simulink model "DRLHevIps"  (R2025b)
settings: Solver=ode23tb  StartTime=0  StopTime=stop_time+1  FixedStep=ts  RelTol=1e-3  AbsTol=1e-4
model workspace (MAT data in the model file):
  BattChrgMax : Simulink.Parameter (value not decoded)
  BattDischrgMax : Simulink.Parameter (value not decoded)
  BrkPrsMax : Simulink.Parameter (value not decoded)
  DiffRatio : Simulink.Parameter (value not decoded)
  EVSpdLmt : Simulink.Parameter (value not decoded)
  EngIdle : Simulink.Parameter (value not decoded)
  EngPwr : Simulink.Parameter (value not decoded)
  EngSpd : Simulink.Parameter (value not decoded)
  EngTrq : Simulink.Parameter (value not decoded)
  EngTrqWhl : Simulink.Parameter (value not decoded)
  GenMapEff : Simulink.Parameter (value not decoded)
  GenMapSpdIndex : Simulink.Parameter (value not decoded)
  GenMapTrqIndex : Simulink.Parameter (value not decoded)
  GenPwrMax : Simulink.Parameter (value not decoded)
  GenSpd : Simulink.Parameter (value not decoded)
  GenTrq : Simulink.Parameter (value not decoded)
  GenTrqMax : Simulink.Parameter (value not decoded)
  MotMapEff : Simulink.Parameter (value not decoded)
  MotMapSpdIndex : Simulink.Parameter (value not decoded)
  MotMapTrqIndex : Simulink.Parameter (value not decoded)
  MotPwr : Simulink.Parameter (value not decoded)
  MotSpd : Simulink.Parameter (value not decoded)
  MotTrq : Simulink.Parameter (value not decoded)
  Ndiff : Simulink.Parameter (value not decoded)
  Nr1 : Simulink.Parameter (value not decoded)
  Nr2 : Simulink.Parameter (value not decoded)
  Ns1 : Simulink.Parameter (value not decoded)
  Ns2 : Simulink.Parameter (value not decoded)
  NsysWhl : Simulink.Parameter (value not decoded)
  SOCChrgFactor : Simulink.Parameter (value not decoded)
  SOCerr : Simulink.Parameter (value not decoded)
  SOCmax : Simulink.Parameter (value not decoded)
  SOCmin : Simulink.Parameter (value not decoded)
  SOCtarget : Simulink.Parameter (value not decoded)
  SysTrqWhl : Simulink.Parameter (value not decoded)
  k : Simulink.Parameter (value not decoded)
values from neighbouring files (symbols this model uses):
  cyc_time = WLTC(:,1)    [mdlrun_time_DG.m]
  cyc_vel = WLTC(:,2)    [mdlrun_time_DG.m]
  en_actsmo = 1    [mdlrun_time_DG.m]
  en_elec = 1    [mdlrun_time_DG.m]
  en_gas = 1    [mdlrun_time_DG.m]
  en_SOCpen = 1    [mdlrun_time_DG.m]
  k_actsmo = 5e-2    (= 0.05)    [mdlrun_time_DG.m]
  k_elec = 1    [mdlrun_time_DG.m]
  k_gas = 1    [mdlrun_time_DG.m]
  k_SOCpen = 1.2    [mdlrun_time_DG.m]
  obs_max = 1e4*[0.0020, 0.0090, 0.0100, 0.0100, 8.4000, 0.0100,                0.0056, 0.1011, 2.8000,      0, 0.0001, 0.0132,                0.0740, 2.6065, 0.0339, 0.0949, 0.0117, 2.4444]    [mdlrun_time_DG.m]
  obs_min = 1e4*[0.0010, 0.0070,      0,      0, 0.8400,      0,                     0, -0.0005,     0, -2.8000,     0, -0.0032               -0.0694, -2.7092, -0.0030,    0, -0.0001, -2.7647]    [mdlrun_time_DG.m]
  Price_elec = 1    [mdlrun_time_DG.m]
  Price_gas = 7.14    [mdlrun_time_DG.m]
  rho_gas = 0.739    [mdlrun_time_DG.m]
  stop_time = cyc_time(end)    [mdlrun_time_DG.m]
  ts = 1    [mdlrun_time_DG.m]
symbols that are objects in the model workspace (value not decoded): BattChrgMax, BattDischrgMax, BrkPrsMax, DiffRatio, EngIdle, EngPwr, EngSpd, EngTrq, EngTrqWhl, EVSpdLmt, GenMapSpdIndex, GenMapTrqIndex, GenPwrMax, GenSpd, GenTrq, GenTrqMax, k, MotMapSpdIndex, MotMapTrqIndex, MotPwr, MotSpd, MotTrq, Ndiff, Nr1, Nr2, Ns1, Ns2, NsysWhl, SOCChrgFactor, SOCerr, SOCmin, SOCtarget, SysTrqWhl
undefined symbols (not defined in the file or in its folder): n_ool, T_ool
libraries: simulink x29, autolibutils x6, slpidlib x2, rllib x2, SignalEditorBlockLib x1, autolibshared x1, autolibhevctrlrcommon x1
(part 3 of 4)

== system DRLHevIps/xCU/xCU/VCU/DRL_Based2_0/DRL action Handle ==
  action : Inport
  EngSpdFdbk : Inport  Port=2
  WhlTrqCmd : Inport  Port=3
  1-D Lookup Table1 : Lookup_n-D  NumberOfTableDimensions=1  BreakpointsForDimension1=[-1, 1]  Table=[n_ool(1), n_ool(end)]  InternalRulePriority=Speed  RndMeth=Simplest
      settings: AttributesFormatString=|
      | %<BreakpointsForDimension1>
      | %<Table>
  1-D Lookup Table2 : Lookup_n-D  NumberOfTableDimensions=1  BreakpointsForDimension1=n_ool  Table=T_ool  InternalRulePriority=Speed  RndMeth=Simplest
      settings: AttributesFormatString=|
      | %<BreakpointsForDimension1>
      | %<Table>
  1-D Lookup Table3 : Lookup_n-D  Commented=on  NumberOfTableDimensions=1  BreakpointsForDimension1=[-1, 1]  Table=[0, max(EngPwr(1,1:15))]  InternalRulePriority=Speed  RndMeth=Simplest
      settings: AttributesFormatString=|
      | %<BreakpointsForDimension1>
      | %<Table>
  Add : Sum  Inputs=-+
  Add1 : Sum
  Add2 : Sum  Inputs=+-
  Gain : Gain  Gain=1/DiffRatio
  Gain1 : Gain  Gain=1/(Nr2/Ns2)
  OptimalEngineSpeed : Lookup_n-D  Commented=on  NumberOfTableDimensions=1  BreakpointsForDimension1=[0 EngPwr(1,1:15)]  Table=[EngIdle*30/pi EngSpd(1,1:15)]  ExtrapMethod=Clip  UseLastTableValue=on  InternalRulePriority=Speed  RndMeth=Simplest
      settings: AttributesFormatString=|
      | %<BreakpointsForDimension1>
      | %<Table>
  OptimalEngineTorque : Lookup_n-D  Commented=on  NumberOfTableDimensions=1  BreakpointsForDimension1=[0 EngPwr(1,1:15)]  Table=[0 EngTrq(1,1:15)]  ExtrapMethod=Clip  UseLastTableValue=on  InternalRulePriority=Speed  RndMeth=Simplest
      settings: AttributesFormatString=|
      | %<BreakpointsForDimension1>
      | %<Table>
  PID Controller : slpidlib/PID Controller  Controller=PI  Form=Parallel  TimeDomain=Discrete-time  UseExternalTs=off  SampleTime=-1  IntegratorMethod=Forward Euler  FilterMethod=Forward Euler  ControllerParametersSource=internal  P=0.18  I=1.0  UseKiTs=off  D=0  UseExternalDerivativeSource=off  N=100  UseFilter=on  TunerSelectOption=Transfer Function Based (PID Tuner App)  InitialConditionSource=internal  InitialConditionForIntegrator=0  InitialConditionForFilter=0  DifferentiatorICPrevScaledInput=0  ExternalReset=none  TrackingMode=off  Kt=1  LimitOutput=on  SatLimitsSource=internal  UpperSaturationLimit=207*42/60-20  LowerSaturationLimit=20-207*42/60  LinearizeAsGain=on  AntiWindupMode=clamping  Kb=1  LimitIntegrator=off  UpperIntegratorSaturationLimit=inf  LowerIntegratorSaturationLimit=-inf  POutMin=[]  POutMax=[]  IOutMin=[]  IOutMax=[]  DOutMin=[]  DOutMax=[]  NOutMin=[]  NOutMax=[]  SumOutMin=[]  SumOutMax=[]  SaturationOutMin=[]  SaturationOutMax=[]  PParamMin=[]  PParamMax=[]  IParamMin=[]  IParamMax=[]  DParamMin=[]  DParamMax=[]  NParamMin=[]  NParamMax=[]  KbParamMin=[]  KbParamMax=[]  KtParamMin=[]  KtParamMax=[]  KbOutMin=[]  KbOutMax=[]  KtOutMin=[]  KtOutMax=[]  IntegratorOutMin=[]  IntegratorOutMax=[]  FilterOutMin=[]  FilterOutMax=[]  SumI1OutMin=[]  SumI1OutMax=[]  SumI2OutMin=[]  SumI2OutMax=[]  SumI3OutMin=[]  SumI3OutMax=[]  SumI4OutMin=[]  SumI4OutMax=[]  SumDOutMin=[]  SumDOutMax=[]  DifferentiatorOutMin=[]  DifferentiatorOutMax=[]  FilterDiffOutCoefMin=[]  FilterDiffOutCoefMax=[]  ReciprocalOutMin=[]  ReciprocalOutMax=[]  SumDenOutMin=[]  SumDenOutMax=[]  SumNumOutMin=[]  SumNumOutMax=[]  DivideOutMin=[]  DivideOutMax=[]  UdiffTsProdOutMin=[]  UdiffTsProdOutMax=[]  NTsProdOutMin=[]  NTsProdOutMax=[]  UintegralTsProdOutMin=[]  UintegralTsProdOutMax=[]  UngainTsProdOutMin=[]  UngainTsProdOutMax=[]  ClampingZeroOutDataTypeStr=Inherit: Inherit via back propagation  ClampingZeroOutMin=[]  ClampingZeroOutMax=[]  FilterDenConstantOutDataTypeStr=Inherit: Inherit via back propagation  FilterDenConstantOutMin=[]  FilterDenConstantOutMax=[]  PCopyOutDataTypeStr=Inherit: Inherit via back propagation  PCopyOutMin=[]  PCopyOutMax=[]  NCopyOutDataTypeStr=Inherit: Inherit via back propagation  NCopyOutMin=[]  NCopyOutMax=[]  IntegratorContinuousStateAttributes=''  IntegratorStateMustResolveToSignalObject=off  IntegratorRTWStateStorageClass=Auto  FilterContinuousStateAttributes=''  FilterStateMustResolveToSignalObject=off  FilterRTWStateStorageClass=Auto  ParallelPVariant=InternalParameters  IdealPVariant=Disabled  IVariant=InternalParameters  DVariant=Disabled  IntegratorVariant=Discrete  SatVariant=Enabled  AWVariant=DiscClampingParallel  PCopyVariant=Disabled  TRVariant=Disabled  FdbkBlocksVariant=Forward  IdealPFdbkVariant=Disabled  SatFdbkVariant=Disabled  DerivativeFilterVariant=Disabled  NVariant=Disabled  NCopyVariant=Disabled_SignalSpec  FilterICVariant=Disabled  IntegratorICVariant=InternalICs  ExternalResetVariant=Disabled  TRSumVariant=Passthrough  SumFdbkVariant=Disabled  SumVariant=Sum_PI  TsampFilterVariant=InternalTs  TsampNgainVariant=Passthrough  TsampIntegralVariant=Disabled_SignalSpec  ExternalSaturationOutDataTypeStr=Inherit: Same as second input  DerivativeSourceVariant=Disabled  PreIntVariant=InternalPreInt
  Product : Product
  Product1 : Product
  Saturation : Saturate  UpperLimit=207*42/60  LowerLimit=-207*42/60
  k1 : Constant  Value=-(1/(1+k))
  k2 : Constant  Value=k/(1+k)
  rads_to_rpm : Gain  Gain=30/pi
  EngTrqCmd : Outport
  GenTrqCmd : Outport  Port=2
  MotTrqCmd : Outport  Port=3
  wires:
  k1/1 -> Product/2
  Add1/1 -> Saturation/1
  WhlTrqCmd/1 -> Gain/1
  k2/1 -> Product1/2
  Product1/1 -> Add/1  "T_e_to_ring"
  Gain/1 -> Add/2  "T_req"
  Add/1 -> Gain1/1
  Product/1 -> Add1/1  "T_g_cmd"
  EngSpdFdbk/1 -> rads_to_rpm/1
  Add2/1 -> PID Controller/1
  PID Controller/1 -> Add1/2
  Saturation/1 -> GenTrqCmd/1
  Gain1/1 -> MotTrqCmd/1  "T_m_cmd"
  rads_to_rpm/1 -> Add2/2
  [EngTrqCmd] -> Product/1
  [EngSpdCmd] -> Add2/1
  [EngTrqCmd] -> Product1/1
  1-D Lookup Table1/1 -> 1-D Lookup Table2/1, [EngSpdCmd]  "w_e_cmd"
  action/1 -> 1-D Lookup Table1/1
  1-D Lookup Table3/1 -> OptimalEngineSpeed/1, OptimalEngineTorque/1
  1-D Lookup Table2/1 -> EngTrqCmd/1, [EngTrqCmd]

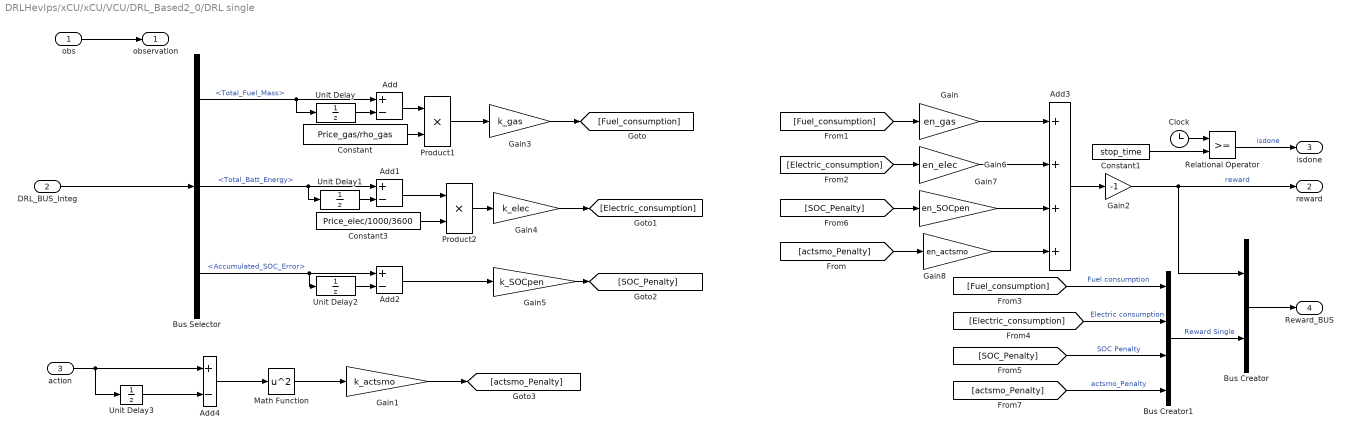
== system DRLHevIps/xCU/xCU/VCU/DRL_Based2_0/DRL single ==
  obs : Inport
  DRL_BUS_Integ : Inport  Port=2
  action : Inport  Port=3
  Add{,1..2,4} (4 alike) : Sum  Inputs=+-
  Add3 : Sum  Inputs=++++
  Bus Creator : BusCreator  Inputs=2
  Bus Creator1 : BusCreator  Inputs=4
  Bus Selector : BusSelector  OutputSignals=Total_Fuel_Mass,Total_Batt_Energy,Accumulated_SOC_Error
  Clock : Clock
  Constant : Constant  Value=Price_gas/rho_gas
  Constant1 : Constant  Value=stop_time
  Constant3 : Constant  Value=Price_elec/1000/3600
  Gain : Gain  Gain=en_gas
  Gain1 : Gain  Gain=k_actsmo
  Gain2 : Gain  Gain=-1
  Gain3 : Gain  Gain=k_gas
  Gain4 : Gain  Gain=k_elec
  Gain5 : Gain  Gain=k_SOCpen
  Gain6 : Gain  Gain=en_elec
  Gain7 : Gain  Gain=en_SOCpen
  Gain8 : Gain  Gain=en_actsmo
  Math Function : Math  Operator=square
  Product1 : Product
  Product2 : Product
  Relational Operator : RelationalOperator  OutDataTypeStr=boolean  RndMeth=Simplest  InputSameDT=off
  Unit Delay : UnitDelay  SampleTime=ts  HasFrameUpgradeWarning=on
  Unit Delay1 : UnitDelay  SampleTime=ts  HasFrameUpgradeWarning=on
  Unit Delay2 : UnitDelay  SampleTime=ts  HasFrameUpgradeWarning=on
  Unit Delay3 : UnitDelay  InitialCondition=-1  SampleTime=ts  HasFrameUpgradeWarning=on
  observation : Outport
  reward : Outport  Port=2
  isdone : Outport  Port=3
  Reward_BUS : Outport  Port=4
  wires:
  [Fuel_consumption] -> Bus Creator1/1  "Fuel consumption"
  [Fuel_consumption] -> Gain/1
  Add3/1 -> Gain2/1
  Gain5/1 -> [SOC_Penalty]
  Constant3/1 -> Product2/2
  Gain3/1 -> [Fuel_consumption]
  [Electric_consumption] -> Bus Creator1/2  "Electric consumption"
  Gain4/1 -> [Electric_consumption]
  Product1/1 -> Gain3/1
  Gain2/1 -> Bus Creator/1, reward/1  "reward"
  Clock/1 -> Relational Operator/1
  [Electric_consumption] -> Gain6/1
  Constant/1 -> Product1/2
  [SOC_Penalty] -> Bus Creator1/3  "SOC Penalty"
  Bus Creator1/1 -> Bus Creator/2  "Reward Single"
  [SOC_Penalty] -> Gain7/1
  Relational Operator/1 -> isdone/1  "isdone"
  Constant1/1 -> Relational Operator/2
  Product2/1 -> Gain4/1
  DRL_BUS_Integ/1 -> Bus Selector/1
  obs/1 -> observation/1
  Bus Selector/1 -> Unit Delay/1, Add/1  "<Total_Fuel_Mass>"
  Unit Delay/1 -> Add/2
  Unit Delay1/1 -> Add1/2
  Bus Selector/2 -> Unit Delay1/1, Add1/1  "<Total_Batt_Energy>"
  Bus Selector/3 -> Unit Delay2/1, Add2/1  "<Accumulated_SOC_Error>"
  Unit Delay2/1 -> Add2/2
  Add1/1 -> Product2/1
  Add/1 -> Product1/1
  Add2/1 -> Gain5/1
  Bus Creator/1 -> Reward_BUS/1
  Unit Delay3/1 -> Add4/2
  action/1 -> Unit Delay3/1, Add4/1
  Add4/1 -> Math Function/1
  Math Function/1 -> Gain1/1
  Gain1/1 -> [actsmo_Penalty]
  [actsmo_Penalty] -> Gain8/1
  [actsmo_Penalty] -> Bus Creator1/4  "actsmo_Penalty"
  Gain/1 -> Add3/1
  Gain6/1 -> Add3/2
  Gain7/1 -> Add3/3
  Gain8/1 -> Add3/4

== system DRLHevIps/xCU/xCU/VCU/DRL_Based2_0/Motor Torque Arbitration and Power Management ==
  MotTrqCmdTrac : Inport
  AccelPed : Inport  Port=2
  BattPwrDisChrgLmt : Inport  Port=3
  "BattPwrChrgLmt " : Inport  Port=4
  GenPwrElec : Inport  Port=5
  MotSpd : Inport  Port=6
  MotTrqCmdRegen : Inport  Port=7
  Accel Decel Switch : Switch  Criteria=u2 > Threshold  SaturateOnIntegerOverflow=off  InputSameDT=off
  Compare To Constant : simulink/Logic and Bit Operations/Compare To Constant  relop=>  const=0  OutDataTypeStr=boolean
  Power Management : Subsystem
  MotTrqCmdFinal : Outport  VectorParamsAs1DForOutWhenUnconnected=off
  wires:
  MotSpd/1 -> Power Management/4(MotSpd)
  "BattPwrChrgLmt "/1 -> Power Management/3(BattPwrChrgLmt)
  GenPwrElec/1 -> Power Management/2(GenPwrElec)
  BattPwrDisChrgLmt/1 -> Power Management/1(BattPwrDischrgLmt)
  Accel Decel Switch/1 -> Power Management/5(MotTrqCmd)
  Power Management/1(MotTrqLim) -> MotTrqCmdFinal/1
  MotTrqCmdTrac/1 -> Accel Decel Switch/1
  Compare To Constant/1 -> Accel Decel Switch/2
  MotTrqCmdRegen/1 -> Accel Decel Switch/3
  AccelPed/1 -> Compare To Constant/1

== system DRLHevIps/xCU/xCU/VCU/DRL_Based2_0/Subsystem ==
  note: T / 4 brakes*(mu*pi*Ba^2*Rm*Npads/4)
  note: 4 brakes*(mu*pi*Ba^2*Rm*Npads/4)*P
  BattSoc : Inport
  VehSpd : Inport  Port=2
  MotSpd : Inport  Port=3
  "BrkPrsReq " : Inport  Port=4
  ChrgLmt : Lookup_n-D  NumberOfTableDimensions=1  BreakpointsForDimension1=[0:10:100]  Table=[1 1 1 1 1 1 1 1 0.7 0.35 0]  ExtrapMethod=Clip  UseLastTableValue=on  InternalRulePriority=Speed  RndMeth=Simplest
  Constant : Constant  Value=4*(0.2*pi*0.05^2*0.1778*2/4)
  Constant1 : Constant  Value=4*(0.2*pi*0.05^2*0.1778*2/4)
  Gain : Gain  Gain=-1
  MaxMotTrqVsSpd : Lookup_n-D  NumberOfTableDimensions=1  BreakpointsForDimension1=MotSpd  Table=MotTrq  ExtrapMethod=Clip  UseLastTableValue=on  InternalRulePriority=Speed  OutDataTypeStr=Inherit: Inherit from 'Table data'  RndMeth=Simplest
  MinMax : MinMax  Inputs=2
  MotTrqReflectedToWheels : Gain  Gain=(Nr2/Ns2)*Ndiff
  Negative 5 : Saturate  UpperLimit=inf  LowerLimit=0
  Product1 : Product
  Product2 : Product
  Product3 : Product
  Product4 : Product  Inputs=*/
  RegenBrakingCutoff : Lookup_n-D  NumberOfTableDimensions=1  BreakpointsForDimension1=[2.2 4.5]  Table=[0 1]  ExtrapMethod=Clip  UseLastTableValue=on  InternalRulePriority=Speed  RndMeth=Simplest
  Subtract : Sum  Inputs=+-
  WhlTrqReflectedToMot : Gain  Gain=1/((Nr2/Ns2)*Ndiff)
  rads_to_rpm : Gain  Gain=30/pi
  " MotTrqCmdRegen" : Outport  VectorParamsAs1DForOutWhenUnconnected=off
  " BrkCmd" : Outport  Port=2  VectorParamsAs1DForOutWhenUnconnected=off
  wires:
  Constant1/1 -> Product4/2
  MotTrqReflectedToWheels/1 -> MinMax/2  "MotTrqMaxWhls"
  Constant/1 -> Product2/2
  BattSoc/1 -> ChrgLmt/1
  ChrgLmt/1 -> Product1/2
  WhlTrqReflectedToMot/1 -> Gain/1
  Product3/1 -> Subtract/2, WhlTrqReflectedToMot/1  "MotTrqRegenWhl"
  Product1/1 -> Product3/2  "RegenFactor"
  Gain/1 -> " MotTrqCmdRegen"/1  "MotTrqCmdRegen"
  rads_to_rpm/1 -> MaxMotTrqVsSpd/1
  Product2/1 -> Subtract/1, MinMax/1  "BrkTrqReqTotal"
  MinMax/1 -> Product3/1  "min"
  MotSpd/1 -> rads_to_rpm/1
  MaxMotTrqVsSpd/1 -> MotTrqReflectedToWheels/1  "MotTrqMax"
  Negative 5/1 -> Product4/1  "BrkTrqFric"
  "BrkPrsReq "/1 -> Product2/1  "BrkPrsReq"
  RegenBrakingCutoff/1 -> Product1/1
  Product4/1 -> " BrkCmd"/1
  Subtract/1 -> Negative 5/1
  VehSpd/1 -> RegenBrakingCutoff/1

== system DRLHevIps/xCU/xCU/VCU/Rule_Based/Accel Pedal to Traction Wheel Torque Request ==
  AccelPed : Inport
  MotSpd : Inport  Port=2
  MaxSysTrqWhlVsWhlSpd : Lookup_n-D  NumberOfTableDimensions=1  BreakpointsForDimension1=NsysWhl  Table=SysTrqWhl  ExtrapMethod=Clip  UseLastTableValue=on  InternalRulePriority=Speed  OutDataTypeStr=Inherit: Inherit from 'Table data'  RndMeth=Simplest
  MotSpdToWhlSpd : Gain  Gain=1/(Nr2/Ns2)/Ndiff
  Product1 : Product
  rads_to_rpm : Gain  Gain=30/pi
  WhlTrqCmd : Outport  VectorParamsAs1DForOutWhenUnconnected=off
  WhlSpd : Outport  Port=2  VectorParamsAs1DForOutWhenUnconnected=off
  wires:
  rads_to_rpm/1 -> MaxSysTrqWhlVsWhlSpd/1
  MotSpdToWhlSpd/1 -> rads_to_rpm/1, WhlSpd/1
  Product1/1 -> WhlTrqCmd/1
  MotSpd/1 -> MotSpdToWhlSpd/1
  MaxSysTrqWhlVsWhlSpd/1 -> Product1/2
  AccelPed/1 -> Product1/1

== system DRLHevIps/xCU/xCU/VCU/Rule_Based/Battery Management System ==
  note: Limit battery charge / discharge power based on SOC
  SOC : Inport
  ChrgLmt : Lookup_n-D  NumberOfTableDimensions=1  BreakpointsForDimension1=[0:10:100]  Table=[1 1 1 1 1 1 1 1 0.7 0.35 0]  ExtrapMethod=Clip  UseLastTableValue=on  InternalRulePriority=Speed  RndMeth=Simplest
  DischrgLmt : Lookup_n-D  NumberOfTableDimensions=1  BreakpointsForDimension1=[0:10:100]  Table=[0 0.35 0.7 1 1 1 1 1 1 1 1]  ExtrapMethod=Clip  UseLastTableValue=on  InternalRulePriority=Speed  RndMeth=Simplest
  MaxChrg : Constant  Value=BattChrgMax
  MaxDischrg : Constant  Value=BattDischrgMax
  Product : Product
  Product1 : Product
  BattPwrDischrgLmt : Outport  VectorParamsAs1DForOutWhenUnconnected=off
  BattPwrChrgLmt : Outport  Port=2  VectorParamsAs1DForOutWhenUnconnected=off
  wires:
  SOC/1 -> DischrgLmt/1, ChrgLmt/1
  MaxChrg/1 -> Product1/2
  MaxDischrg/1 -> Product/2
  Product/1 -> BattPwrDischrgLmt/1
  Product1/1 -> BattPwrChrgLmt/1
  ChrgLmt/1 -> Product1/1
  DischrgLmt/1 -> Product/1

== system DRLHevIps/xCU/xCU/VCU/Rule_Based/Brake Pedal to Total Braking Pressure Request ==
  Brk : Inport
  Park : Inport  Port=2
  Constant : Constant  Value=BrkPrsMax
  Constant1 : Constant  Value=0.5
  Product1 : Product
  Switch : Switch  Criteria=u2 > Threshold  SaturateOnIntegerOverflow=off  InputSameDT=off
  BrkPrsReq : Outport  VectorParamsAs1DForOutWhenUnconnected=off
  wires:
  Constant/1 -> Product1/2
  Product1/1 -> BrkPrsReq/1
  Switch/1 -> Product1/1
  Brk/1 -> Switch/3
  Park/1 -> Switch/2
  Constant1/1 -> Switch/1

== system DRLHevIps/xCU/xCU/VCU/Rule_Based/Motor Torque Arbitration and Power Management ==
  MotTrqCmdTrac : Inport
  AccelPed : Inport  Port=2
  BattPwrDisChrgLmt : Inport  Port=3
  "BattPwrChrgLmt " : Inport  Port=4
  GenPwrElec : Inport  Port=5
  MotSpd : Inport  Port=6
  MotTrqCmdRegen : Inport  Port=7
  Accel Decel Switch : Switch  Criteria=u2 > Threshold  SaturateOnIntegerOverflow=off  InputSameDT=off
  Compare To Constant : simulink/Logic and Bit Operations/Compare To Constant  relop=>  const=0  OutDataTypeStr=boolean
  Power Management : Subsystem
  MotTrqCmdFinal : Outport  VectorParamsAs1DForOutWhenUnconnected=off
  wires:
  AccelPed/1 -> Compare To Constant/1
  MotTrqCmdRegen/1 -> Accel Decel Switch/3
  Compare To Constant/1 -> Accel Decel Switch/2
  MotTrqCmdTrac/1 -> Accel Decel Switch/1
  Power Management/1(MotTrqLim) -> MotTrqCmdFinal/1
  Accel Decel Switch/1 -> Power Management/5(MotTrqCmd)
  BattPwrDisChrgLmt/1 -> Power Management/1(BattPwrDischrgLmt)
  GenPwrElec/1 -> Power Management/2(GenPwrElec)
  "BattPwrChrgLmt "/1 -> Power Management/3(BattPwrChrgLmt)
  MotSpd/1 -> Power Management/4(MotSpd)

== system DRLHevIps/xCU/xCU/VCU/Rule_Based/Subsystem ==
  note: 4 brakes*(mu*pi*Ba^2*Rm*Npads/4)*P
  note: T / 4 brakes*(mu*pi*Ba^2*Rm*Npads/4)
  BattSoc : Inport
  VehSpd : Inport  Port=2
  MotSpd : Inport  Port=3
  "BrkPrsReq " : Inport  Port=4
  ChrgLmt : Lookup_n-D  NumberOfTableDimensions=1  BreakpointsForDimension1=[0:10:100]  Table=[1 1 1 1 1 1 1 1 0.7 0.35 0]  ExtrapMethod=Clip  UseLastTableValue=on  InternalRulePriority=Speed  RndMeth=Simplest
  Constant : Constant  Value=4*(0.2*pi*0.05^2*0.1778*2/4)
  Constant1 : Constant  Value=4*(0.2*pi*0.05^2*0.1778*2/4)
  Gain : Gain  Gain=-1
  MaxMotTrqVsSpd : Lookup_n-D  NumberOfTableDimensions=1  BreakpointsForDimension1=MotSpd  Table=MotTrq  ExtrapMethod=Clip  UseLastTableValue=on  InternalRulePriority=Speed  OutDataTypeStr=Inherit: Inherit from 'Table data'  RndMeth=Simplest
  MinMax : MinMax  Inputs=2
  MotTrqReflectedToWheels : Gain  Gain=(Nr2/Ns2)*Ndiff
  Negative 5 : Saturate  UpperLimit=inf  LowerLimit=0
  Product1 : Product
  Product2 : Product
  Product3 : Product
  Product4 : Product  Inputs=*/
  RegenBrakingCutoff : Lookup_n-D  NumberOfTableDimensions=1  BreakpointsForDimension1=[2.2 4.5]  Table=[0 1]  ExtrapMethod=Clip  UseLastTableValue=on  InternalRulePriority=Speed  RndMeth=Simplest
  Subtract : Sum  Inputs=+-
  WhlTrqReflectedToMot : Gain  Gain=1/((Nr2/Ns2)*Ndiff)
  rads_to_rpm : Gain  Gain=30/pi
  " MotTrqCmdRegen" : Outport  VectorParamsAs1DForOutWhenUnconnected=off
  " BrkCmd" : Outport  Port=2  VectorParamsAs1DForOutWhenUnconnected=off
  wires:
  VehSpd/1 -> RegenBrakingCutoff/1
  Subtract/1 -> Negative 5/1
  Product4/1 -> " BrkCmd"/1
  RegenBrakingCutoff/1 -> Product1/1
  "BrkPrsReq "/1 -> Product2/1  "BrkPrsReq"
  Negative 5/1 -> Product4/1  "BrkTrqFric"
  MaxMotTrqVsSpd/1 -> MotTrqReflectedToWheels/1  "MotTrqMax"
  MotSpd/1 -> rads_to_rpm/1
  MinMax/1 -> Product3/1  "min"
  Product2/1 -> MinMax/1, Subtract/1  "BrkTrqReqTotal"
  rads_to_rpm/1 -> MaxMotTrqVsSpd/1
  Gain/1 -> " MotTrqCmdRegen"/1  "MotTrqCmdRegen"
  Product1/1 -> Product3/2  "RegenFactor"
  Product3/1 -> WhlTrqReflectedToMot/1, Subtract/2  "MotTrqRegenWhl"
  WhlTrqReflectedToMot/1 -> Gain/1
  ChrgLmt/1 -> Product1/2
  BattSoc/1 -> ChrgLmt/1
  Constant/1 -> Product2/2
  MotTrqReflectedToWheels/1 -> MinMax/2  "MotTrqMaxWhls"
  Constant1/1 -> Product4/2

== system DRLHevIps/xCU/xCU/VCU/Rule_Based_DataGen/Accel Pedal to Traction Wheel Torque Request ==
  AccelPed : Inport
  MotSpd : Inport  Port=2
  MaxSysTrqWhlVsWhlSpd : Lookup_n-D  NumberOfTableDimensions=1  BreakpointsForDimension1=NsysWhl  Table=SysTrqWhl  ExtrapMethod=Clip  UseLastTableValue=on  InternalRulePriority=Speed  OutDataTypeStr=Inherit: Inherit from 'Table data'  RndMeth=Simplest
  MotSpdToWhlSpd : Gain  Gain=1/(Nr2/Ns2)/Ndiff
  Product1 : Product
  rads_to_rpm : Gain  Gain=30/pi
  WhlTrqCmd : Outport  VectorParamsAs1DForOutWhenUnconnected=off
  WhlSpd : Outport  Port=2  VectorParamsAs1DForOutWhenUnconnected=off
  wires:
  rads_to_rpm/1 -> MaxSysTrqWhlVsWhlSpd/1
  MotSpdToWhlSpd/1 -> rads_to_rpm/1, WhlSpd/1
  Product1/1 -> WhlTrqCmd/1
  MotSpd/1 -> MotSpdToWhlSpd/1
  MaxSysTrqWhlVsWhlSpd/1 -> Product1/2
  AccelPed/1 -> Product1/1

== system DRLHevIps/xCU/xCU/VCU/Rule_Based_DataGen/Battery Management System ==
  note: Limit battery charge / discharge power based on SOC
  SOC : Inport
  ChrgLmt : Lookup_n-D  NumberOfTableDimensions=1  BreakpointsForDimension1=[0:10:100]  Table=[1 1 1 1 1 1 1 1 0.7 0.35 0]  ExtrapMethod=Clip  UseLastTableValue=on  InternalRulePriority=Speed  RndMeth=Simplest
  DischrgLmt : Lookup_n-D  NumberOfTableDimensions=1  BreakpointsForDimension1=[0:10:100]  Table=[0 0.35 0.7 1 1 1 1 1 1 1 1]  ExtrapMethod=Clip  UseLastTableValue=on  InternalRulePriority=Speed  RndMeth=Simplest
  MaxChrg : Constant  Value=BattChrgMax
  MaxDischrg : Constant  Value=BattDischrgMax
  Product : Product
  Product1 : Product
  BattPwrDischrgLmt : Outport  VectorParamsAs1DForOutWhenUnconnected=off
  BattPwrChrgLmt : Outport  Port=2  VectorParamsAs1DForOutWhenUnconnected=off
  wires:
  SOC/1 -> DischrgLmt/1, ChrgLmt/1
  MaxChrg/1 -> Product1/2
  MaxDischrg/1 -> Product/2
  Product/1 -> BattPwrDischrgLmt/1
  Product1/1 -> BattPwrChrgLmt/1
  ChrgLmt/1 -> Product1/1
  DischrgLmt/1 -> Product/1

== system DRLHevIps/xCU/xCU/VCU/Rule_Based_DataGen/Brake Pedal to Total Braking Pressure Request ==
  Brk : Inport
  Park : Inport  Port=2
  Constant : Constant  Value=BrkPrsMax
  Constant1 : Constant  Value=0.5
  Product1 : Product
  Switch : Switch  Criteria=u2 > Threshold  SaturateOnIntegerOverflow=off  InputSameDT=off
  BrkPrsReq : Outport  VectorParamsAs1DForOutWhenUnconnected=off
  wires:
  Constant/1 -> Product1/2
  Product1/1 -> BrkPrsReq/1
  Switch/1 -> Product1/1
  Brk/1 -> Switch/3
  Park/1 -> Switch/2
  Constant1/1 -> Switch/1

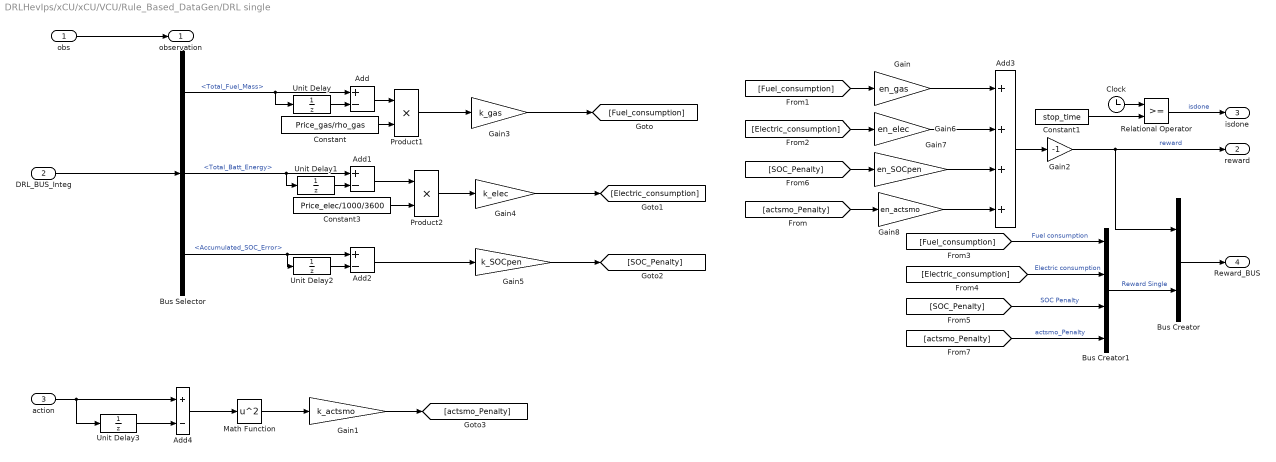
== system DRLHevIps/xCU/xCU/VCU/Rule_Based_DataGen/DRL single ==
  obs : Inport
  DRL_BUS_Integ : Inport  Port=2
  action : Inport  Port=3
  Add{,1..2,4} (4 alike) : Sum  Inputs=+-
  Add3 : Sum  Inputs=++++
  Bus Creator : BusCreator  Inputs=2
  Bus Creator1 : BusCreator  Inputs=4
  Bus Selector : BusSelector  OutputSignals=Total_Fuel_Mass,Total_Batt_Energy,Accumulated_SOC_Error
  Clock : Clock
  Constant : Constant  Value=Price_gas/rho_gas
  Constant1 : Constant  Value=stop_time
  Constant3 : Constant  Value=Price_elec/1000/3600
  Gain : Gain  Gain=en_gas
  Gain1 : Gain  Gain=k_actsmo
  Gain2 : Gain  Gain=-1
  Gain3 : Gain  Gain=k_gas
  Gain4 : Gain  Gain=k_elec
  Gain5 : Gain  Gain=k_SOCpen
  Gain6 : Gain  Gain=en_elec
  Gain7 : Gain  Gain=en_SOCpen
  Gain8 : Gain  Gain=en_actsmo
  Math Function : Math  Operator=square
  Product1 : Product
  Product2 : Product
  Relational Operator : RelationalOperator  OutDataTypeStr=boolean  RndMeth=Simplest  InputSameDT=off
  Unit Delay : UnitDelay  SampleTime=ts  HasFrameUpgradeWarning=on
  Unit Delay1 : UnitDelay  SampleTime=ts  HasFrameUpgradeWarning=on
  Unit Delay2 : UnitDelay  SampleTime=ts  HasFrameUpgradeWarning=on
  Unit Delay3 : UnitDelay  InitialCondition=-1  SampleTime=ts  HasFrameUpgradeWarning=on
  observation : Outport
  reward : Outport  Port=2
  isdone : Outport  Port=3
  Reward_BUS : Outport  Port=4
  wires:
  [Fuel_consumption] -> Bus Creator1/1  "Fuel consumption"
  [Fuel_consumption] -> Gain/1
  Add3/1 -> Gain2/1
  Gain5/1 -> [SOC_Penalty]
  Constant3/1 -> Product2/2
  Gain3/1 -> [Fuel_consumption]
  [Electric_consumption] -> Bus Creator1/2  "Electric consumption"
  Gain4/1 -> [Electric_consumption]
  Product1/1 -> Gain3/1
  Gain2/1 -> Bus Creator/1, reward/1  "reward"
  Clock/1 -> Relational Operator/1
  [Electric_consumption] -> Gain6/1
  Constant/1 -> Product1/2
  [SOC_Penalty] -> Bus Creator1/3  "SOC Penalty"
  Bus Creator1/1 -> Bus Creator/2  "Reward Single"
  [SOC_Penalty] -> Gain7/1
  Relational Operator/1 -> isdone/1  "isdone"
  Constant1/1 -> Relational Operator/2
  Product2/1 -> Gain4/1
  DRL_BUS_Integ/1 -> Bus Selector/1
  obs/1 -> observation/1
  Bus Selector/1 -> Unit Delay/1, Add/1  "<Total_Fuel_Mass>"
  Unit Delay/1 -> Add/2
  Unit Delay1/1 -> Add1/2
  Bus Selector/2 -> Unit Delay1/1, Add1/1  "<Total_Batt_Energy>"
  Bus Selector/3 -> Unit Delay2/1, Add2/1  "<Accumulated_SOC_Error>"
  Unit Delay2/1 -> Add2/2
  Add1/1 -> Product2/1
  Add/1 -> Product1/1
  Add2/1 -> Gain5/1
  Bus Creator/1 -> Reward_BUS/1
  Unit Delay3/1 -> Add4/2
  action/1 -> Unit Delay3/1, Add4/1
  Add4/1 -> Math Function/1
  Math Function/1 -> Gain1/1
  Gain1/1 -> [actsmo_Penalty]
  [actsmo_Penalty] -> Gain8/1
  [actsmo_Penalty] -> Bus Creator1/4  "actsmo_Penalty"
  Gain/1 -> Add3/1
  Gain6/1 -> Add3/2
  Gain7/1 -> Add3/3
  Gain8/1 -> Add3/4

== system DRLHevIps/xCU/xCU/VCU/Rule_Based_DataGen/HevIps Supervisory Control/Engine_Control.Run.TrqCalc ==
  EngPwrCmd : Inport  OutDataTypeStr=double  PortDimensions=1
  f : TriggerPort  TriggerType=function-call  VariantControl=Variant  StatesWhenEnabling=reset
      settings: CopyFcn=Stateflow.SLINSF.SimulinkMan.removeBlockPreDeleteFcn  PreDeleteFcn=Stateflow.SLINSF.SimulinkMan.unsafePredeleteFcn
  OptimalEngineSpeed : Lookup_n-D  NumberOfTableDimensions=1  BreakpointsForDimension1=[0 EngPwr(1,1:15)]  Table=[EngIdle*30/pi EngSpd(1,1:15)]  ExtrapMethod=Clip  UseLastTableValue=on  InternalRulePriority=Speed  RndMeth=Simplest
      settings: AttributesFormatString=|
      | %<BreakpointsForDimension1>
      | %<Table>
  OptimalEngineTorque : Lookup_n-D  NumberOfTableDimensions=1  BreakpointsForDimension1=[0 EngPwr(1,1:15)]  Table=[0 EngTrq(1,1:15)]  ExtrapMethod=Clip  UseLastTableValue=on  InternalRulePriority=Speed  RndMeth=Simplest
      settings: AttributesFormatString=|
      | %<BreakpointsForDimension1>
      | %<Table>
  rpm_to_rads : Gain  Gain=pi/30
  EngTrqCmd : Outport  VectorParamsAs1DForOutWhenUnconnected=off
  EngSpdCmd : Outport  Port=2  VectorParamsAs1DForOutWhenUnconnected=off
  wires:
  OptimalEngineTorque/1 -> EngTrqCmd/1
  OptimalEngineSpeed/1 -> rpm_to_rads/1
  rpm_to_rads/1 -> EngSpdCmd/1
  EngPwrCmd/1 -> OptimalEngineSpeed/1, OptimalEngineTorque/1

== system DRLHevIps/xCU/xCU/VCU/Rule_Based_DataGen/HevIps Supervisory Control/Generator_Control.ON.GenControl ==
  note: OutLim
  GenSpd : Inport  OutDataTypeStr=double  PortDimensions=1
  EngSpd : Inport  Port=2  OutDataTypeStr=double  PortDimensions=1
  BattPwrDischrgLmt : Inport  Port=3  OutDataTypeStr=double  PortDimensions=1
  MotPwrElec : Inport  Port=4  OutDataTypeStr=double  PortDimensions=1
  BattPwrChrgLmt : Inport  Port=5  OutDataTypeStr=double  PortDimensions=1
  EngSpdCmd : Inport  Port=6  OutDataTypeStr=double  PortDimensions=1
  EngMode : Inport  Port=7  OutDataTypeStr=double  PortDimensions=1
  f : TriggerPort  TriggerType=function-call  VariantControl=Variant  StatesWhenEnabling=reset  SampleTime=-1
      settings: CopyFcn=Stateflow.SLINSF.SimulinkMan.removeBlockPreDeleteFcn  PreDeleteFcn=Stateflow.SLINSF.SimulinkMan.unsafePredeleteFcn
  Compare To Constant : simulink/Logic and Bit Operations/Compare To Constant  relop===  const=3  OutDataTypeStr=boolean
  Constant : Constant  Value=GenTrqMax
  Constant1 : Constant  Value=max(EngTrq)*Ns1/(Nr1+Ns1)
  Gain : Gain  Gain=-1
  PID Controller1 : slpidlib/PID Controller  Controller=PI  Form=Parallel  TimeDomain=Discrete-time  UseExternalTs=off  SampleTime=-1  IntegratorMethod=Forward Euler  FilterMethod=Forward Euler  ControllerParametersSource=internal  P=1  I=3  UseKiTs=off  D=1  UseExternalDerivativeSource=off  N=100  UseFilter=on  TunerSelectOption=Transfer Function Based (PID Tuner App)  ZeroCross=off  InitialConditionSource=internal  InitialConditionForIntegrator=0  InitialConditionForFilter=0  DifferentiatorICPrevScaledInput=0  ExternalReset=none  TrackingMode=off  Kt=1  LimitOutput=on  SatLimitsSource=internal  UpperSaturationLimit=GenTrqMax  LowerSaturationLimit=-GenTrqMax  LinearizeAsGain=on  AntiWindupMode=clamping  Kb=1  LimitIntegrator=off  UpperIntegratorSaturationLimit=inf  LowerIntegratorSaturationLimit=-inf  POutMin=[]  POutMax=[]  IOutMin=[]  IOutMax=[]  DOutMin=[]  DOutMax=[]  NOutMin=[]  NOutMax=[]  SumOutMin=[]  SumOutMax=[]  SaturationOutMin=[]  SaturationOutMax=[]  PParamMin=[]  PParamMax=[]  IParamMin=[]  IParamMax=[]  DParamMin=[]  DParamMax=[]  NParamMin=[]  NParamMax=[]  KbParamMin=[]  KbParamMax=[]  KtParamMin=[]  KtParamMax=[]  KbOutMin=[]  KbOutMax=[]  KtOutMin=[]  KtOutMax=[]  IntegratorOutMin=[]  IntegratorOutMax=[]  FilterOutMin=[]  FilterOutMax=[]  SumI1OutMin=[]  SumI1OutMax=[]  SumI2OutMin=[]  SumI2OutMax=[]  SumI3OutMin=[]  SumI3OutMax=[]  SumI4OutMin=[]  SumI4OutMax=[]  SumDOutMin=[]  SumDOutMax=[]  DifferentiatorOutMin=[]  DifferentiatorOutMax=[]  FilterDiffOutCoefMin=[]  FilterDiffOutCoefMax=[]  ReciprocalOutMin=[]  ReciprocalOutMax=[]  SumDenOutMin=[]  SumDenOutMax=[]  SumNumOutMin=[]  SumNumOutMax=[]  DivideOutMin=[]  DivideOutMax=[]  UdiffTsProdOutMin=[]  UdiffTsProdOutMax=[]  NTsProdOutMin=[]  NTsProdOutMax=[]  UintegralTsProdOutMin=[]  UintegralTsProdOutMax=[]  UngainTsProdOutMin=[]  UngainTsProdOutMax=[]  ClampingZeroOutDataTypeStr=Inherit: Inherit via back propagation  ClampingZeroOutMin=[]  ClampingZeroOutMax=[]  FilterDenConstantOutDataTypeStr=Inherit: Inherit via back propagation  FilterDenConstantOutMin=[]  FilterDenConstantOutMax=[]  PCopyOutDataTypeStr=Inherit: Inherit via back propagation  PCopyOutMin=[]  PCopyOutMax=[]  NCopyOutDataTypeStr=Inherit: Inherit via back propagation  NCopyOutMin=[]  NCopyOutMax=[]  IntegratorContinuousStateAttributes=''  IntegratorStateMustResolveToSignalObject=off  IntegratorRTWStateStorageClass=Auto  FilterContinuousStateAttributes=''  FilterStateMustResolveToSignalObject=off  FilterRTWStateStorageClass=Auto  ParallelPVariant=InternalParameters  IdealPVariant=Disabled  IVariant=InternalParameters  DVariant=Disabled  IntegratorVariant=Discrete  SatVariant=Enabled  AWVariant=DiscClampingParallel  PCopyVariant=Disabled  TRVariant=Disabled  FdbkBlocksVariant=Forward  IdealPFdbkVariant=Disabled  SatFdbkVariant=Disabled  DerivativeFilterVariant=Disabled  NVariant=Disabled  NCopyVariant=Disabled_SignalSpec  FilterICVariant=Disabled  IntegratorICVariant=InternalICs  ExternalResetVariant=Disabled  TRSumVariant=Passthrough  SumFdbkVariant=Disabled  SumVariant=Sum_PI  TsampFilterVariant=InternalTs  TsampNgainVariant=Passthrough  TsampIntegralVariant=Disabled_SignalSpec  ExternalSaturationOutDataTypeStr=Inherit: Same as second input  DerivativeSourceVariant=Disabled  PreIntVariant=InternalPreInt
  Power Management : Subsystem
  Saturation Dynamic1 : simulink/Discontinuities/Saturation Dynamic  OutMin=[]  OutMax=[]  OutDataTypeStr=Inherit: Same as second input  OutDataType=fixdt(1, 16)  OutScaling=2^-10  DoSatur=off
  Subtract2 : Sum  Inputs=+-
  Switch : Switch  Criteria=u2 > Threshold  SaturateOnIntegerOverflow=off  InputSameDT=off
  EngSpdErr : Outport  VectorParamsAs1DForOutWhenUnconnected=off
  GenTrqCmd : Outport  Port=2  VectorParamsAs1DForOutWhenUnconnected=off
  GenPwrCmd : Outport  Port=3  VectorParamsAs1DForOutWhenUnconnected=off
  wires:
  [Out] -> Power Management/1(GenTrqCmdPI)
  PID Controller1/1 -> [PI]
  Power Management/2(GenPwrCmd) -> GenPwrCmd/1
  Power Management/1(GenTrqCmd) -> GenTrqCmd/1
  EngMode/1 -> [EngMode], Power Management/6(EngMode)
  EngSpdCmd/1 -> Subtract2/1
  GenSpd/1 -> Power Management/2(GenSpd)
  BattPwrChrgLmt/1 -> Power Management/5(BattPwrChrgLmt)
  BattPwrDischrgLmt/1 -> Power Management/3(BattPwrDischrgLmt)
  MotPwrElec/1 -> Power Management/4(MotPwrElec)
  EngSpd/1 -> Subtract2/2
  Subtract2/1 -> EngSpdErr/1, PID Controller1/1
  Saturation Dynamic1/1 -> [Out]
  Compare To Constant/1 -> Switch/2
  Gain/1 -> Saturation Dynamic1/3
  [PI] -> Saturation Dynamic1/2
  [EngMode] -> Compare To Constant/1
  Switch/1 -> Saturation Dynamic1/1, Gain/1
  Constant/1 -> Switch/3
  Constant1/1 -> Switch/1

== system DRLHevIps/xCU/xCU/VCU/Rule_Based_DataGen/HevIps Supervisory Control/Motor_Control.Mot_EV.MotTrqEV ==
  WhlTrqCmd : Inport  OutDataTypeStr=double  PortDimensions=1
  f : TriggerPort  TriggerType=function-call  VariantControl=Variant  StatesWhenEnabling=reset
      settings: CopyFcn=Stateflow.SLINSF.SimulinkMan.removeBlockPreDeleteFcn  PreDeleteFcn=Stateflow.SLINSF.SimulinkMan.unsafePredeleteFcn
  WhlTrqReflectedMotTrq : Gain  Gain=1/(Nr2/Ns2)/Ndiff
  MotTrqCmd : Outport  VectorParamsAs1DForOutWhenUnconnected=off
  wires:
  WhlTrqReflectedMotTrq/1 -> MotTrqCmd/1
  WhlTrqCmd/1 -> WhlTrqReflectedMotTrq/1

== system DRLHevIps/xCU/xCU/VCU/Rule_Based_DataGen/HevIps Supervisory Control/Motor_Control.Mot_HEV.MotTrqHEV ==
  MotPwrCmd : Inport  OutDataTypeStr=double  PortDimensions=1
  MotSpd : Inport  Port=2  OutDataTypeStr=double  PortDimensions=1
  f : TriggerPort  TriggerType=function-call  VariantControl=Variant  StatesWhenEnabling=reset
      settings: CopyFcn=Stateflow.SLINSF.SimulinkMan.removeBlockPreDeleteFcn  PreDeleteFcn=Stateflow.SLINSF.SimulinkMan.unsafePredeleteFcn
  Elec_to_MechPwr1 : Product  Inputs=*/
  div0protect - poly : autolibutils/div0protect - poly  thresh=2  ZeroCross1=off  aMode=aMode
  MotTrqCmd : Outport  VectorParamsAs1DForOutWhenUnconnected=off
  wires:
  Elec_to_MechPwr1/1 -> MotTrqCmd/1
  div0protect - poly/1 -> Elec_to_MechPwr1/2
  MotSpd/1 -> div0protect - poly/1
  MotPwrCmd/1 -> Elec_to_MechPwr1/1

== system DRLHevIps/xCU/xCU/VCU/Rule_Based_DataGen/HevIps Supervisory Control/Operating_Modes.Driving.HEV.High_Power_Charge_Deplete.OpMode4 ==
  note: EngPwrCmd = WhlPwrCmd (up to EngPwrMax)
      | MotPwrCmd =  (WhlTrqCmd - EngTrqCmd_Wheels)*WhlSpd
  WhlTrqCmd : Inport  OutDataTypeStr=double  PortDimensions=1
  WhlSpd : Inport  Port=2  OutDataTypeStr=double  PortDimensions=1
  WhlPwrCmd : Inport  Port=3  OutDataTypeStr=double  PortDimensions=1
  EngTrqOut : Inport  Port=4  OutDataTypeStr=double  PortDimensions=1
  f : TriggerPort  TriggerType=function-call  VariantControl=Variant  StatesWhenEnabling=reset
      settings: CopyFcn=Stateflow.SLINSF.SimulinkMan.removeBlockPreDeleteFcn  PreDeleteFcn=Stateflow.SLINSF.SimulinkMan.unsafePredeleteFcn
  CarrierTrqToRingTrg : Gain  Gain=Nr1/(Nr1+Ns1)
  Product1 : Product
  RingTrqToMot : Gain  Gain=Ns2/Nr2
  RingTrqToWhlTrq : Gain  Gain=Ndiff
  Saturation : Saturate  UpperLimit=max(EngPwr(1,1:15))  LowerLimit=0
      settings: AttributesFormatString=[%<LowerLimit>, %<UpperLimit>]
  Saturation1 : Saturate  UpperLimit=inf  LowerLimit=0
      settings: AttributesFormatString=[%<LowerLimit>, %<UpperLimit>]
  Saturation4 : Saturate  UpperLimit=max(MotPwr)  LowerLimit=0
      settings: AttributesFormatString=[%<LowerLimit>, %<UpperLimit>]
  Sum2 : Sum  Inputs=+-
  Terminator1 : Terminator
  WhlTrqToRingTrq : Gain  Gain=1/Ndiff
  EngPwrCmd : Outport  VectorParamsAs1DForOutWhenUnconnected=off
  MotPwrCmd : Outport  Port=2  VectorParamsAs1DForOutWhenUnconnected=off
  wires:
  Saturation4/1 -> MotPwrCmd/1
  WhlPwrCmd/1 -> Saturation/1
  Saturation/1 -> EngPwrCmd/1
  EngTrqOut/1 -> CarrierTrqToRingTrg/1
  Product1/1 -> Saturation4/1  "MotPwrAssist"
  RingTrqToMot/1 -> Terminator1/1  "MotTrqAssist"
  WhlTrqToRingTrq/1 -> RingTrqToMot/1
  Saturation1/1 -> Product1/1, WhlTrqToRingTrq/1
  Sum2/1 -> Saturation1/1
  RingTrqToWhlTrq/1 -> Sum2/2
  WhlTrqCmd/1 -> Sum2/1
  WhlSpd/1 -> Product1/2
  CarrierTrqToRingTrg/1 -> RingTrqToWhlTrq/1

== system DRLHevIps/xCU/xCU/VCU/Rule_Based_DataGen/HevIps Supervisory Control/Operating_Modes.Driving.HEV.Low_Power_Charge_Sustain.OpMode3 ==
  note: Torque Blending
  note: EngPwrCmd = WhlPwrCmd + ChargePwr
      | MotPwrCmd = GenPwrCmd - ChargePwr
  note: 当发电机消耗正功率时限制充电。
  note: 此功能在从电动模式（使用电机）过渡至低功率模式（使用发动机）时，协调动力系统扭矩的平滑转换。它允许电机根据发动机扭矩的上升而逐渐降低其扭矩输出。一旦混合过程完成，如有需要，电机可启动其维持充电状态（负扭矩）。
  WhlPwrCmd : Inport  OutDataTypeStr=double  PortDimensions=1
  ChrgPwr : Inport  Port=2  OutDataTypeStr=double  PortDimensions=1
  BattPwrChrgLmt : Inport  Port=3  OutDataTypeStr=double  PortDimensions=1
  GenPwrCmd : Inport  Port=4  OutDataTypeStr=double  PortDimensions=1
  EngTrqOut : Inport  Port=5  OutDataTypeStr=double  PortDimensions=1
  EngSpd : Inport  Port=6  OutDataTypeStr=double  PortDimensions=1
  f : TriggerPort  TriggerType=function-call  VariantControl=Variant  StatesWhenEnabling=reset
      settings: CopyFcn=Stateflow.SLINSF.SimulinkMan.removeBlockPreDeleteFcn  PreDeleteFcn=Stateflow.SLINSF.SimulinkMan.unsafePredeleteFcn
  Constant : Constant  Value=0
  Gain1 : Gain  Gain=-1
  LPF IC : autolibutils/LPF IC  w=10  aMode=aMode  dataType=off
  Product2 : Product
  Saturation : Saturate  UpperLimit=max(EngPwr(1,1:15))  LowerLimit=0
      settings: AttributesFormatString=[%<LowerLimit>, %<UpperLimit>]
  Saturation Dynamic3 : simulink/Discontinuities/Saturation Dynamic  OutMin=[]  OutMax=[]  OutDataTypeStr=Inherit: Same as second input  OutDataType=fixdt(1, 16)  OutScaling=2^-10  DoSatur=off
  Saturation3 : Saturate  UpperLimit=0  LowerLimit=-GenPwrMax
      settings: AttributesFormatString=[%<LowerLimit>, %<UpperLimit>]
  Saturation5 : Saturate  UpperLimit=inf  LowerLimit=0
      settings: AttributesFormatString=[%<LowerLimit>, %<UpperLimit>]
  Sum1 : Sum  Inputs=-+
  Sum3 : Sum
  Sum6 : Sum  Inputs=+-
  Switch : Switch  SaturateOnIntegerOverflow=off  InputSameDT=off
  Unary Minus1 : UnaryMinus
  EngPwrCmd : Outport  VectorParamsAs1DForOutWhenUnconnected=off
  MotPwrCmd : Outport  Port=2  VectorParamsAs1DForOutWhenUnconnected=off
  wires:
  LPF IC/1 -> MotPwrCmd/1
  Sum1/1 -> [MotPwrLow]
  Saturation3/1 -> Sum1/2
  WhlPwrCmd/1 -> [WhlPwrCmd], Sum3/1
  Constant/1 -> Saturation Dynamic3/3
  BattPwrChrgLmt/1 -> Unary Minus1/1
  Gain1/1 -> Saturation3/1
  GenPwrCmd/1 -> Gain1/1
  Saturation Dynamic3/1 -> Sum3/2, Sum1/1
  Saturation/1 -> EngPwrCmd/1
  ChrgPwr/1 -> Saturation Dynamic3/2
  Sum3/1 -> Saturation/1
  Unary Minus1/1 -> Saturation Dynamic3/1
  [MotPwrLow] -> Switch/3
  Sum6/1 -> Switch/2, Saturation5/1
  EngTrqOut/1 -> Product2/1
  Saturation5/1 -> Switch/1
  Product2/1 -> Sum6/2  "EngPwrOut"
  EngSpd/1 -> Product2/2
  [WhlPwrCmd] -> Sum6/1
  Switch/1 -> LPF IC/2, LPF IC/1

== system DRLHevIps/xCU/xCU/VCU/Rule_Based_DataGen/HevIps Supervisory Control/Operating_Modes.Driving.HEV.ModeSelection ==
  note: RelayDynLowLimit
  note: 此功能通过车轮的Power命令和AccCmd来确定使用低速模式还是高速模式。
  note: Relay Logic w/ Dynamic Lower Limit
  WhlSpd : Inport  OutDataTypeStr=double  PortDimensions=1
  WhlPwrCmd : Inport  Port=2  OutDataTypeStr=double  PortDimensions=1
  AccelPed : Inport  Port=3  OutDataTypeStr=double  PortDimensions=1
  ChrgPwr : Inport  Port=4  OutDataTypeStr=double  PortDimensions=1
  BattPwrChrgLmt : Inport  Port=5  OutDataTypeStr=double  PortDimensions=1
  f : TriggerPort  TriggerType=function-call  VariantControl=Variant  StatesWhenEnabling=reset
      settings: CopyFcn=Stateflow.SLINSF.SimulinkMan.removeBlockPreDeleteFcn  PreDeleteFcn=Stateflow.SLINSF.SimulinkMan.unsafePredeleteFcn
  Add1 : Sum  Inputs=-+
  Compare To Constant : simulink/Logic and Bit Operations/Compare To Constant  relop===  const=1  OutDataTypeStr=boolean
  Compare To Constant1 : simulink/Logic and Bit Operations/Compare To Constant  relop===  const=1  OutDataTypeStr=boolean
  Compare To Constant2 : simulink/Logic and Bit Operations/Compare To Constant  relop===  const=0  OutDataTypeStr=boolean
  Constant : Constant  Value=0
  Logical Operator : Logic  AllPortsSameDT=off  OutDataTypeStr=boolean
  Logical Operator1 : Logic  Operator=OR  AllPortsSameDT=off  OutDataTypeStr=boolean
  Logical Operator2 : Logic  Operator=NOT  AllPortsSameDT=off  OutDataTypeStr=boolean
  Logical Operator3 : Logic  AllPortsSameDT=off  OutDataTypeStr=boolean
  OptimalEngineTorqueAtWheels : Lookup_n-D  NumberOfTableDimensions=1  BreakpointsForDimension1=NsysWhl  Table=EngTrqWhl  ExtrapMethod=Clip  UseLastTableValue=on  InternalRulePriority=Speed  RndMeth=Simplest
      settings: AttributesFormatString=|
      | %<BreakpointsForDimension1>
      | %<Table>
  Product : Product
  Relational Operator : RelationalOperator  Operator=>  OutDataTypeStr=boolean  RndMeth=Simplest  InputSameDT=off
  Relational Operator1 : RelationalOperator  Operator=<  OutDataTypeStr=boolean  RndMeth=Simplest  InputSameDT=off
  Saturation Dynamic3 : simulink/Discontinuities/Saturation Dynamic  OutMin=[]  OutMax=[]  OutDataTypeStr=Inherit: Same as second input  OutDataType=fixdt(1, 16)  OutScaling=2^-10  DoSatur=off
  Switch : Switch  Criteria=u2 > Threshold  SaturateOnIntegerOverflow=off  InputSameDT=off
  Switch1 : Switch  Criteria=u2 > Threshold  SaturateOnIntegerOverflow=off  InputSameDT=off
  Unary Minus1 : UnaryMinus
  Unary Minus2 : UnaryMinus
  Unit Delay : UnitDelay  SampleTime=-1  HasFrameUpgradeWarning=on
  Upper Limit : Constant  Value=0
  off : Constant  Value=0  OutDataTypeStr=boolean
  on : Constant  OutDataTypeStr=boolean
  rads_to_rpm : Gain  Gain=30/pi
  Low : Outport  VectorParamsAs1DForOutWhenUnconnected=off
  High : Outport  Port=2  VectorParamsAs1DForOutWhenUnconnected=off
  wires:
  AccelPed/1 -> Compare To Constant/1
  Switch/1 -> Unit Delay/1, Logical Operator1/1
  Logical Operator2/1 -> Low/1
  WhlPwrCmd/1 -> Add1/2
  Saturation Dynamic3/1 -> Unary Minus2/1
  Unary Minus1/1 -> Saturation Dynamic3/1
  ChrgPwr/1 -> Saturation Dynamic3/2
  BattPwrChrgLmt/1 -> Unary Minus1/1
  Constant/1 -> Saturation Dynamic3/3
  Product/1 -> Add1/1  "EngPwrWhls"
  Logical Operator1/1 -> High/1, Logical Operator2/1
  Compare To Constant/1 -> Logical Operator1/2
  OptimalEngineTorqueAtWheels/1 -> Product/1
  rads_to_rpm/1 -> OptimalEngineTorqueAtWheels/1
  WhlSpd/1 -> Product/2, rads_to_rpm/1
  Add1/1 -> Relational Operator1/1, Relational Operator/1
  Upper Limit/1 -> Relational Operator/2
  Unary Minus2/1 -> Relational Operator1/2
  Relational Operator/1 -> Logical Operator/1
  Compare To Constant2/1 -> Logical Operator/2
  Relational Operator1/1 -> Logical Operator3/1
  Compare To Constant1/1 -> Logical Operator3/2
  Logical Operator/1 -> Switch/2
  on/1 -> Switch/1
  Logical Operator3/1 -> Switch1/2
  off/1 -> Switch1/1
  Switch1/1 -> Switch/3
  Unit Delay/1 -> Compare To Constant2/1, Compare To Constant1/1, Switch1/3

== system DRLHevIps/xCU/xCU/VCU/Rule_Based_DataGen/HevIps Supervisory Control/Operating_Modes.EngOnCalc ==
  note: Check Power
  note: If Pbatt > PlimBattDischrg
      | for > 0.1 sec, turn EngOn
  SOC : Inport  OutDataTypeStr=double  PortDimensions=1
  BattPwr : Inport  Port=2  OutDataTypeStr=double  PortDimensions=1
  BattPwrDischrgLmt : Inport  Port=3  OutDataTypeStr=double  PortDimensions=1
  VehSpd : Inport  Port=4  OutDataTypeStr=double  PortDimensions=1
  EVSpdLmt : Inport  Port=5  OutDataTypeStr=double  PortDimensions=1
  AccelPed : Inport  Port=6  OutDataTypeStr=double  PortDimensions=1
  WhlPwrCmd : Inport  Port=7  OutDataTypeStr=double  PortDimensions=1
  SOCopt : Inport  Port=8  OutDataTypeStr=double  PortDimensions=1
  OpMode : Inport  Port=9  OutDataTypeStr=double  PortDimensions=1
  f : TriggerPort  TriggerType=function-call  VariantControl=Variant  StatesWhenEnabling=reset
      settings: CopyFcn=Stateflow.SLINSF.SimulinkMan.removeBlockPreDeleteFcn  PreDeleteFcn=Stateflow.SLINSF.SimulinkMan.unsafePredeleteFcn
  1-D Lookup Table : Lookup_n-D  NumberOfTableDimensions=1  BreakpointsForDimension1=[55 70]  Table=[EngPwr(1) EngPwr(2)]  ExtrapMethod=Clip  UseLastTableValue=on  InternalRulePriority=Speed  RndMeth=Simplest
      settings: AttributesFormatString=|
      | %<BreakpointsForDimension1>
      | %<Table>
  Compare To Constant : simulink/Logic and Bit Operations/Compare To Constant  relop=>  const=0.9  OutDataTypeStr=boolean
  Compare To Constant1 : simulink/Logic and Bit Operations/Compare To Constant  relop===  const=6  OutDataTypeStr=boolean
  Gain : Gain  Gain=100
  Logical Operator : Logic  Operator=OR  Inputs=6  AllPortsSameDT=off  OutDataTypeStr=boolean
  Logical Operator1 : Logic  AllPortsSameDT=off  OutDataTypeStr=boolean
  Relational Operator : RelationalOperator  Operator=>  OutDataTypeStr=boolean  RndMeth=Simplest  InputSameDT=off
  Relational Operator1 : RelationalOperator  Operator=<  OutDataTypeStr=boolean  RndMeth=Simplest  InputSameDT=off
  Relational Operator2 : RelationalOperator  Operator=>  OutDataTypeStr=boolean  RndMeth=Simplest  InputSameDT=off
  Relational Operator3 : RelationalOperator  OutDataTypeStr=boolean  RndMeth=Simplest  InputSameDT=off
  Timer : Stateflow chart  TreatAsAtomicUnit=on
  EngOnReq : Outport  VectorParamsAs1DForOutWhenUnconnected=off
  wires:
  Gain/1 -> Relational Operator1/2
  WhlPwrCmd/1 -> Relational Operator/1
  Relational Operator1/1 -> Logical Operator/2
  Compare To Constant1/1 -> Logical Operator/6
  OpMode/1 -> Compare To Constant1/1
  SOCopt/1 -> Gain/1
  1-D Lookup Table/1 -> Relational Operator/2
  Relational Operator/1 -> Logical Operator/1
  SOC/1 -> Relational Operator1/1, 1-D Lookup Table/1
  Compare To Constant/1 -> Logical Operator/3
  AccelPed/1 -> Compare To Constant/1
  VehSpd/1 -> Relational Operator2/1
  EVSpdLmt/1 -> Relational Operator2/2
  Relational Operator2/1 -> Logical Operator/4
  Logical Operator/1 -> EngOnReq/1
  Logical Operator1/1 -> Logical Operator/5
  Timer/1(Out) -> Logical Operator1/2
  BattPwrDischrgLmt/1 -> Relational Operator3/2
  BattPwr/1 -> Relational Operator3/1
  Relational Operator3/1 -> Logical Operator1/1, Timer/1(In)

== system DRLHevIps/xCU/xCU/VCU/Rule_Based_DataGen/HevIps Supervisory Control/Operating_Modes.Stationary.Charging.ChargePowerCalc ==
  SOC : Inport  OutDataTypeStr=double  PortDimensions=1
  f : TriggerPort  TriggerType=function-call  VariantControl=Variant  StatesWhenEnabling=reset
      settings: CopyFcn=Stateflow.SLINSF.SimulinkMan.removeBlockPreDeleteFcn  PreDeleteFcn=Stateflow.SLINSF.SimulinkMan.unsafePredeleteFcn
  Charge Power : Lookup_n-D  NumberOfTableDimensions=1  BreakpointsForDimension1=[20 SOCtarget]  Table=[20000 0]  ExtrapMethod=Clip  UseLastTableValue=on  InternalRulePriority=Speed  RndMeth=Simplest
      settings: AttributesFormatString=|
      | %<BreakpointsForDimension1>
      | %<Table>
  EngPwrCmd : Outport  VectorParamsAs1DForOutWhenUnconnected=off
  wires:
  Charge Power/1 -> EngPwrCmd/1
  SOC/1 -> Charge Power/1

== system DRLHevIps/xCU/xCU/VCU/Rule_Based_DataGen/Motor Torque Arbitration and Power Management ==
  MotTrqCmdTrac : Inport
  AccelPed : Inport  Port=2
  BattPwrDisChrgLmt : Inport  Port=3
  "BattPwrChrgLmt " : Inport  Port=4
  GenPwrElec : Inport  Port=5
  MotSpd : Inport  Port=6
  MotTrqCmdRegen : Inport  Port=7
  Accel Decel Switch : Switch  Criteria=u2 > Threshold  SaturateOnIntegerOverflow=off  InputSameDT=off
  Compare To Constant : simulink/Logic and Bit Operations/Compare To Constant  relop=>  const=0  OutDataTypeStr=boolean
  Power Management : Subsystem
  MotTrqCmdFinal : Outport  VectorParamsAs1DForOutWhenUnconnected=off
  wires:
  AccelPed/1 -> Compare To Constant/1
  MotTrqCmdRegen/1 -> Accel Decel Switch/3
  Compare To Constant/1 -> Accel Decel Switch/2
  MotTrqCmdTrac/1 -> Accel Decel Switch/1
  Power Management/1(MotTrqLim) -> MotTrqCmdFinal/1
  Accel Decel Switch/1 -> Power Management/5(MotTrqCmd)
  BattPwrDisChrgLmt/1 -> Power Management/1(BattPwrDischrgLmt)
  GenPwrElec/1 -> Power Management/2(GenPwrElec)
  "BattPwrChrgLmt "/1 -> Power Management/3(BattPwrChrgLmt)
  MotSpd/1 -> Power Management/4(MotSpd)
